simulink model "reorder_double_buffer_test"  (Simulink 7.2)
settings: Solver=VariableStepDiscrete  StartTime=0.0  StopTime=200  RelTol=1e-3
libraries: xbsIndex_r4 x30, casper_library_reorder x2, casper_library_delays x1
settings Model: Creator=User  LastModifiedBy=root
settings OptimizationCC: InitFltsAndDblsToZero=on
settings DebuggingCC: SaveWithDisabledLinksMsg=none  SaveWithParameterizedLinksMsg=none

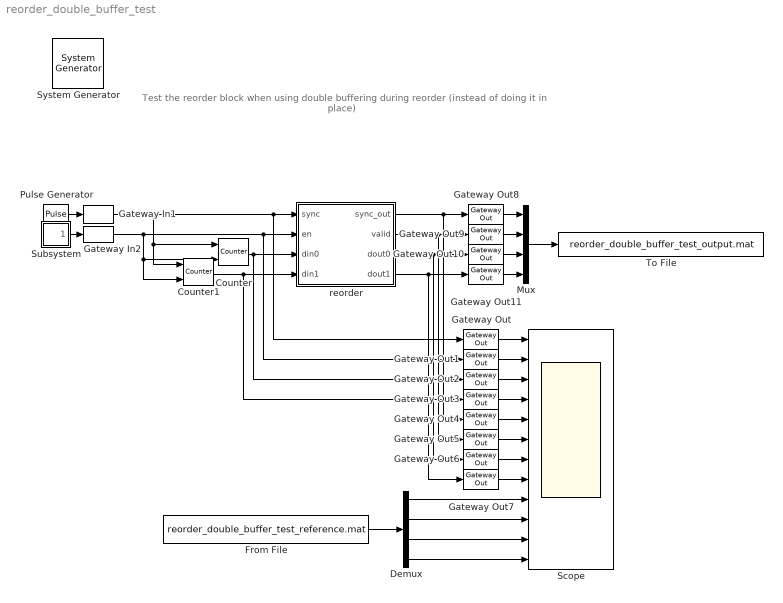
== system reorder_double_buffer_test ==
  note: Test the reorder block when
      | using double buffering during
      | reorder (instead of doing
      | it in place)
  " System Generator" : xbsIndex_r4/ System Generator  Tag=genX  SystemSampleTime=-1  xilinxfamily=Virtex4  part=xc4vsx35  speed=-10  package=ff668  synthesis_tool=XST  clock_wrapper=Clock Enables  directory=./netlist  testbench=off  simulink_period=1  sysclk_period=100  dcm_input_clock_period=100  incr_netlist=off  trim_vbits=Everywhere in SubSystem  dbl_ovrd=According to Block Masks  core_generation=According to Block Masks  run_coregen=off  deprecated_control=off  eval_field=0  block_type=sysgen
      settings: block_version=10.1.1
  Counter : xbsIndex_r4/Counter  cnt_type=Free Running  cnt_to=Inf  operation=Up  start_count=0  cnt_by_val=1  arith_type=Unsigned  n_bits=3  bin_pt=0  load_pin=off  rst=on  en=on  explicit_period=on  period=1  dbl_ovrd=off  use_behavioral_HDL=off  implementation=Fabric  block_type=counter
      settings: block_version=11.4
  Counter1 : xbsIndex_r4/Counter  cnt_type=Free Running  cnt_to=Inf  operation=Down  start_count=0  cnt_by_val=1  arith_type=Unsigned  n_bits=3  bin_pt=0  load_pin=off  rst=on  en=on  explicit_period=on  period=1  dbl_ovrd=off  use_behavioral_HDL=off  implementation=Fabric  block_type=counter
      settings: block_version=11.4
  Demux : Demux
  From File : FromFile  FileName=reorder_double_buffer_test_reference.mat  SampleTime=1
  Gateway In1 : xbsIndex_r4/Gateway In  arith_type=Boolean  n_bits=16  bin_pt=14  quantization="Round  (unbiased: +/- Inf)"  overflow=Saturate  period=1  dbl_ovrd=off  timing_constraint=None  locs_specified=off  LOCs={}  hdl_port=on  block_type=gatewayin
      settings: infoedit="Gateway in block.  Converts inputs of type Simulink integer, double and fixed point to  Xilinx fixed point type.<P><P>Hardware notes:  In hardware these blocks become top level input ports."  block_version=10.1.1
  Gateway In2 : xbsIndex_r4/Gateway In  arith_type=Boolean  n_bits=16  bin_pt=14  quantization="Round  (unbiased: +/- Inf)"  overflow=Saturate  period=1  dbl_ovrd=off  timing_constraint=None  locs_specified=off  LOCs={}  hdl_port=on  block_type=gatewayin
      settings: infoedit="Gateway in block.  Converts inputs of type Simulink integer, double and fixed point to  Xilinx fixed point type.<P><P>Hardware notes:  In hardware these blocks become top level input ports."  block_version=10.1.1
  Gateway Out{,1..11} (12 alike) : xbsIndex_r4/Gateway Out  hdl_port=on  timing_constraint=None  locs_specified=off  LOCs={}  block_type=gatewayout
      settings: infoedit="Gateway out block.  Converts Xilinx fixed point inputs into ouputs of type Simulink integer, double, or fixed point.<P><P>Hardware notes:  In hardware these blocks become top level output ports or are discarded, depending on how they are configured."  block_version=10.1.1
  Mux : Mux
  Pulse Generator : DiscretePulseGenerator  Period=64  PhaseDelay=13
  Scope : Scope  NumInputPorts=12
      settings: TimeRange=37.32833957553058  YMin=0~0~-50~-50~0~0~-50~-50~0~0~-6.382978723404449~-50  YMax=1~1~50~50~1~1~50~50~1~1~40.42553191489355~50
  Subsystem : Subsystem
  To File : ToFile  Filename=reorder_double_buffer_test_output.mat  MatrixName=output
  reorder : Subsystem  AncestorBlock=casper_library_reorder/reorder  mask(reorder){map=getfield( getfield( get_param( gcb,'UserData' ), 'parameters'),'map'), n_inputs=2, bram_latency=2, map_latency=2, double_buffer=1, bram_map=off}
      mask prompts: map "Output Order:"; n_inputs "Number of inputs"; bram_latency "BRAM Latency"; map_latency "Map Latency"; double_buffer "Double Buffer"; bram_map "Use BlockRAM for Map"
      mask init:
      | reorder_init(gcb, ...
      |     'map', map, ...
      |     'n_inputs', n_inputs, ...
      |     'bram_latency', bram_latency, ...
      |     'map_latency', map_latency, ...
      |     'double_buffer', double_buffer, ...
      |     'bram_map', bram_map);
      settings: AttributesFormatString=order=2
      mask Help: eval('xlWeb(''http://casper.berkeley.edu/wiki/Reorder'')')
  wires:
  Pulse Generator/1 -> Gateway In1/1
  Subsystem/1(Out1) -> Gateway In2/1
  Gateway In1/1 -> Gateway Out/1, reorder/1(sync), Counter/1, Counter1/1
  Gateway In2/1 -> Gateway Out1/1, reorder/2(en), Counter/2, Counter1/2
  Counter/1 -> Gateway Out2/1, reorder/3(din0)
  Counter1/1 -> Gateway Out3/1, reorder/4(din1)
  Gateway Out/1 -> Scope/1
  Gateway Out1/1 -> Scope/2
  Gateway Out2/1 -> Scope/3
  Gateway Out3/1 -> Scope/4
  reorder/1(sync_out) -> Gateway Out4/1, Gateway Out8/1
  reorder/2(valid) -> Gateway Out5/1, Gateway Out9/1
  reorder/3(dout0) -> Gateway Out6/1, Gateway Out10/1
  reorder/4(dout1) -> Gateway Out7/1, Gateway Out11/1
  Gateway Out4/1 -> Scope/5
  Gateway Out5/1 -> Scope/6
  Gateway Out6/1 -> Scope/7
  Gateway Out7/1 -> Scope/8
  Mux/1 -> To File/1
  From File/1 -> Demux/1
  Demux/1 -> Scope/9
  Demux/2 -> Scope/10
  Demux/3 -> Scope/11
  Demux/4 -> Scope/12
  Gateway Out8/1 -> Mux/1
  Gateway Out11/1 -> Mux/4
  Gateway Out10/1 -> Mux/3
  Gateway Out9/1 -> Mux/2

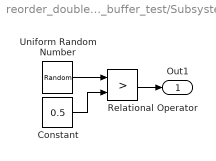
== system reorder_double_buffer_test/Subsystem ==
  Constant : Constant  Value=0.5  OutDataType=sfix(16)  OutScaling=2^0
  Relational Operator : RelationalOperator  Operator=>  LogicOutDataTypeMode=boolean  OutDataTypeStr=boolean
  Uniform Random Number : UniformRandomNumber  Minimum=0  SampleTime=1
  Out1 : Outport
  wires:
  Uniform Random Number/1 -> Relational Operator/1
  Constant/1 -> Relational Operator/2
  Relational Operator/1 -> Out1/1

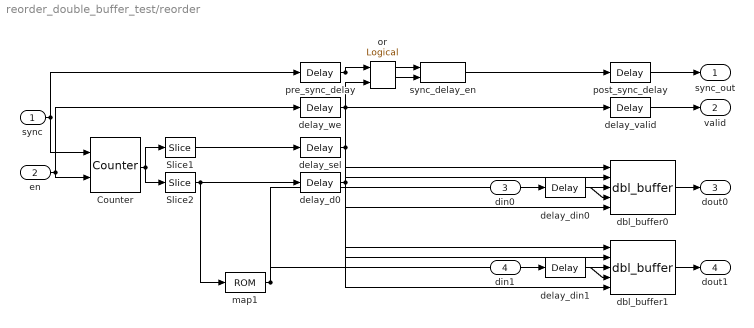
== system reorder_double_buffer_test/reorder ==
  sync : Inport  OutDataType=sfix(16)  OutScaling=2^0
  en : Inport  Port=2  OutDataType=sfix(16)  OutScaling=2^0
  din0 : Inport  Port=3  OutDataType=sfix(16)  OutScaling=2^0
  din1 : Inport  Port=4  OutDataType=sfix(16)  OutScaling=2^0
  Counter : xbsIndex_r4/Counter  cnt_type=Count Limited  cnt_to=15  operation=Up  start_count=0  cnt_by_val=1  arith_type=Unsigned  n_bits=4  bin_pt=0  load_pin=off  rst=on  en=on  explicit_period=on  period=1  dbl_ovrd=off  use_behavioral_HDL=off  implementation=Fabric  block_type=counter
      settings: block_version=11.4
  Slice1 : xbsIndex_r4/Slice  nbits=1  boolean_output=off  mode=Upper Bit Location + Width  bit1=0  base1=MSB of Input  bit0=0  base0=LSB of Input  dbl_ovrd=off  block_type=slice
  Slice2 : xbsIndex_r4/Slice  nbits=3  boolean_output=off  mode=Lower Bit Location + Width  bit1=0  base1=MSB of Input  bit0=0  base0=LSB of Input  dbl_ovrd=off  block_type=slice
  dbl_buffer0 : casper_library_reorder/dbl_buffer  SystemSampleTime=-1  depth=8  latency=2
  dbl_buffer1 : casper_library_reorder/dbl_buffer  SystemSampleTime=-1  depth=8  latency=2
  delay_d0 : xbsIndex_r4/Delay  en=off  latency=2  dbl_ovrd=off  reg_retiming=off  block_type=delay
      settings: block_version=11.4
  delay_din0 : xbsIndex_r4/Delay  en=off  latency=2  dbl_ovrd=off  reg_retiming=off  block_type=delay
      settings: xl_area=[0, 0, 0, 0, 0, 0, 0]  block_version=9.1.01
  delay_din1 : xbsIndex_r4/Delay  en=off  latency=2  dbl_ovrd=off  reg_retiming=off  block_type=delay
      settings: xl_area=[0, 0, 0, 0, 0, 0, 0]  block_version=9.1.01
  delay_sel : xbsIndex_r4/Delay  en=off  latency=2  dbl_ovrd=off  reg_retiming=off  block_type=delay
      settings: block_version=11.4
  delay_valid : xbsIndex_r4/Delay  en=off  latency=4  dbl_ovrd=off  reg_retiming=off  block_type=delay
      settings: xl_area=[0, 0, 0, 0, 0, 0, 0]  block_version=9.1.01
  delay_we : xbsIndex_r4/Delay  en=off  latency=2  dbl_ovrd=off  reg_retiming=off  block_type=delay
      settings: xl_area=[0, 0, 0, 0, 0, 0, 0]  block_version=9.1.01
  map1 : xbsIndex_r4/ROM  depth=8  initVector=map  distributed_mem=Distributed memory  rst=off  init_reg=0  en=off  latency=2  arith_type=Unsigned  n_bits=3  bin_pt=0  dbl_ovrd=off  optimize=Area  use_rpm=on  block_type=sprom
      settings: block_version=11.4
  or : xbsIndex_r4/Logical  logical_function=OR  inputs=2  en=off  latency=0  precision=Full  arith_type=Unsigned  n_bits=16  bin_pt=0  align_bp=on  dbl_ovrd=off  block_type=logical
      settings: block_version=11.4
  post_sync_delay : xbsIndex_r4/Delay  en=off  latency=4  dbl_ovrd=off  reg_retiming=off  block_type=delay
      settings: block_version=11.4
  pre_sync_delay : xbsIndex_r4/Delay  en=off  latency=2  dbl_ovrd=off  reg_retiming=off  block_type=delay
      settings: block_version=11.4
  sync_delay_en : casper_library_delays/sync_delay_en  SystemSampleTime=-1  DelayLen=8
  sync_out : Outport  OutDataType=sfix(16)  OutScaling=2^0
  valid : Outport  Port=2  OutDataType=sfix(16)  OutScaling=2^0
  dout0 : Outport  Port=3  OutDataType=sfix(16)  OutScaling=2^0
  dout1 : Outport  Port=4  OutDataType=sfix(16)  OutScaling=2^0
  wires:
  en/1 -> delay_we/1, Counter/2
  delay_we/1 -> delay_valid/1, or/2, dbl_buffer0/5, dbl_buffer1/5
  delay_valid/1 -> valid/1
  sync/1 -> pre_sync_delay/1, Counter/1
  pre_sync_delay/1 -> or/1, sync_delay_en/1
  or/1 -> sync_delay_en/2
  sync_delay_en/1 -> post_sync_delay/1
  post_sync_delay/1 -> sync_out/1
  Counter/1 -> Slice1/1, Slice2/1
  Slice1/1 -> delay_sel/1
  Slice2/1 -> delay_d0/1, map1/1
  delay_d0/1 -> dbl_buffer0/2, dbl_buffer1/2
  map1/1 -> dbl_buffer0/3, dbl_buffer1/3
  delay_sel/1 -> dbl_buffer0/1, dbl_buffer1/1
  din0/1 -> delay_din0/1
  delay_din0/1 -> dbl_buffer0/4
  dbl_buffer0/1 -> dout0/1
  din1/1 -> delay_din1/1
  delay_din1/1 -> dbl_buffer1/4
  dbl_buffer1/1 -> dout1/1
